simulink model "PerceptionAndGuidance"  (R2026b)
settings: Solver=ode3  StopTime=TFinal
PreLoadFcn:
  | InitVars;
libraries: simulink x3, visiongeotforms x3, raspberrypiAVlib x2, raspberrypiutilitieslib x2, raspberrypiCommlib x2
settings Model: Creator=The MathWorks, Inc.  LastModifiedBy=Deepak Vishwakarma
settings SolverCC: AutoInsertRateTranBlk=on  PositivePriorityOrder=on
settings OptimizationCC: DifferentSizesBufferReuse=on  EfficientTunableParamExpr=on  EnhancedBackFolding=on  MaxStackSize=200000  OptimizationCustomize=off  OptimizeBlockOrder=speed  PassReuseOutputArgsAs=Individual arguments  RemoveInternalMemoryZeroInit=on  RemoveRootLevelIOMemoryZeroInit=on
settings DebuggingCC: ParameterPrecisionLossMsg=none  ParameterTunabilityLossMsg=error
settings HardwareCC: ProdHWDeviceType=ARM Compatible->ARM Cortex-A (32-bit)  ProdLargestAtomicFloat=Double  ProdLargestAtomicInteger=Long  ProdLongLongMode=on
settings ModelReferenceCC: PropagateVarSize=During execution
settings RTWCC: BuildConfiguration=Faster Runs  Description=Embedded Coder  HardwareBoard=Raspberry Pi  SystemTargetFile=ert.tlc  TLCOptions="-aInlineSetEventsForThisBaseRateFcn=TLC_FALSE -aSuppressMultiTaskScheduler=TLC_FALSE  -aRateBasedStepFcn=0"  TemplateMakefile=ert_default_tmf  Toolchain=GNU GCC RPIUtils
settings CodeAppCC: ForceParamTrailComments=on  IgnoreCustomStorageClasses=off  InsertBlockDesc=on  OperatorAnnotations=on  SFDataObjDesc=on  SimulinkDataObjDesc=on
settings ERTTargetCC: CodeReplacementLibrary=ARM Cortex-A CMSIS  ExtModeIntrfLevel=Level2 - Open  ExtModeMexFile=ext_xcp  ExtModeStaticAlloc=on  SupportVariableSizeSignals=on

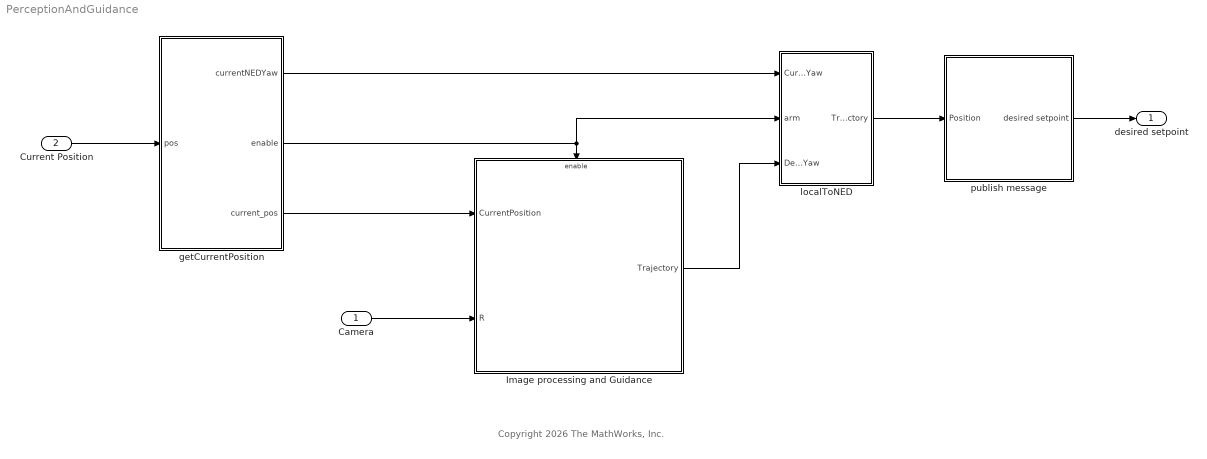
== system PerceptionAndGuidance ==
  note: Copyright 2026 The MathWorks, Inc.
  Camera : Inport
  Current Position : Inport  Port=2
  Image processing and Guidance : Subsystem
  getCurrentPosition : Subsystem  Variant=on
  localToNED : Subsystem
  publish message : Subsystem  Variant=on
  desired setpoint : Outport  OutDataTypeStr=Bus: desiredTargetSetpoints
  wires:
  localToNED/1(Trajectory) -> publish message/1(Position)
  getCurrentPosition/1(currentNEDYaw) -> localToNED/1(CurrentNEDYaw)
  Image processing and Guidance/1(Trajectory) -> localToNED/3(DesiredPosAndYaw)
  getCurrentPosition/2(enable) -> Image processing and Guidance/Enable, localToNED/2(arm)
  Camera/1 -> Image processing and Guidance/2(R)
  Current Position/1 -> getCurrentPosition/1(pos)
  getCurrentPosition/3(current_pos) -> Image processing and Guidance/1(CurrentPosition)
  publish message/1(desired setpoint) -> desired setpoint/1

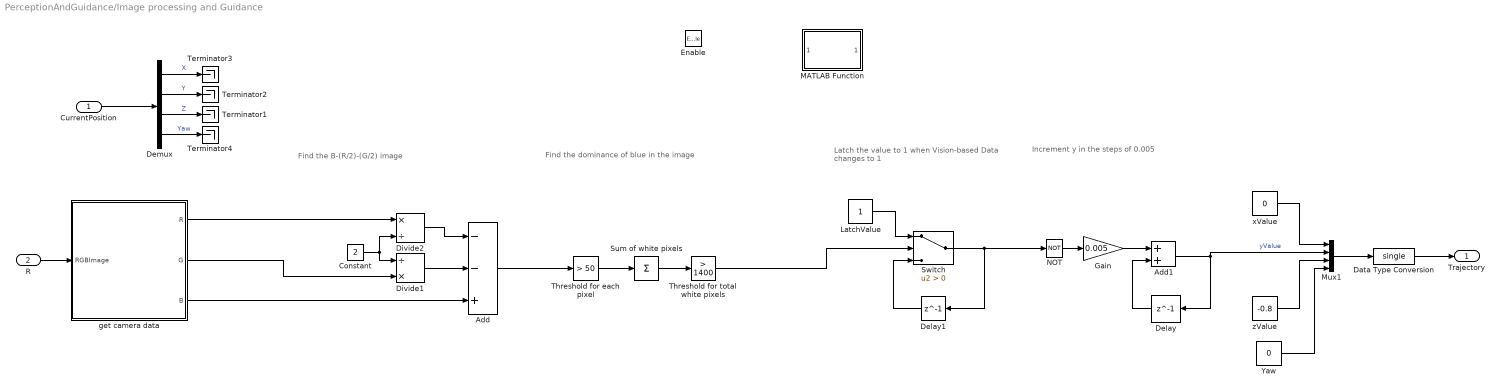
== system PerceptionAndGuidance/Image processing and Guidance ==
  note: Find the dominance of blue in the image
  note: Increment y in the steps of 0.005
  note: Find the B-(R/2)-(G/2) image
  note: Latch the value to 1 when
      | Vision-based Data changes to 1
  CurrentPosition : Inport
  R : Inport  Port=2
  Enable : EnablePort
  Add : Sum  Inputs=--+
  Add1 : Sum
  Constant : Constant  Value=2  SampleTime=-1
  Data Type Conversion : DataTypeConversion  OutDataTypeStr=single  SaturateOnIntegerOverflow=off  RndMeth=Floor
  Delay : Delay  DelayLength=1
  Delay1 : Delay  DelayLength=1
  Demux : Demux
  Divide1 : Product  Inputs=/*
  Divide2 : Product  Inputs=*/
  Gain : Gain  Gain=0.005
  LatchValue : Constant  SampleTime=-1
  MATLAB Function : MATLAB Function  TreatAsAtomicUnit=on
  Mux1 : Mux
  NOT : Logic  Operator=NOT  IconShape=distinctive  AllPortsSameDT=off  OutDataTypeStr=boolean
  Sum of white pixels : Sum  Inputs=+  OutDataTypeStr=uint16
  Switch : Switch  Criteria=u2 > Threshold  SaturateOnIntegerOverflow=off  InputSameDT=off
  Terminator{1..4} (4 alike) : Terminator
  Threshold for each pixel : simulink/Logic and Bit Operations/Compare To Constant  relop=>  const=50  OutDataTypeStr=boolean
  Threshold for total white pixels : simulink/Logic and Bit Operations/Compare To Constant  relop=>  const=1400  OutDataTypeStr=boolean
  Yaw : Constant  Value=0  OutDataTypeStr=double  SampleTime=-1
  get camera data : Subsystem  Variant=on
  xValue : Constant  Value=0  SampleTime=-1
  zValue : Constant  Value=-0.8  SampleTime=-1
  Trajectory : Outport
  wires:
  NOT/1 -> Gain/1
  Divide2/1 -> Add/1
  zValue/1 -> Mux1/3
  Sum of white pixels/1 -> Threshold for total white pixels/1
  get camera data/1(R) -> Divide2/1
  LatchValue/1 -> Switch/1
  Threshold for total white pixels/1 -> Switch/2
  R/1 -> get camera data/1(RGBImage)
  Add1/1 -> Delay/1, Mux1/2  "yValue"
  Constant/1 -> Divide1/1, Divide2/2
  Divide1/1 -> Add/2
  Switch/1 -> NOT/1, Delay1/1
  Delay1/1 -> Switch/3
  Gain/1 -> Add1/1
  Threshold for each pixel/1 -> Sum of white pixels/1
  Delay/1 -> Add1/2
  get camera data/2(G) -> Divide1/2
  Add/1 -> Threshold for each pixel/1
  xValue/1 -> Mux1/1
  get camera data/3(B) -> Add/3
  Data Type Conversion/1 -> Trajectory/1
  Yaw/1 -> Mux1/4
  Mux1/1 -> Data Type Conversion/1
  CurrentPosition/1 -> Demux/1
  Demux/4 -> Terminator4/1  "Yaw"
  Demux/3 -> Terminator1/1  "Z"
  Demux/2 -> Terminator2/1  "Y"
  Demux/1 -> Terminator3/1  "X"

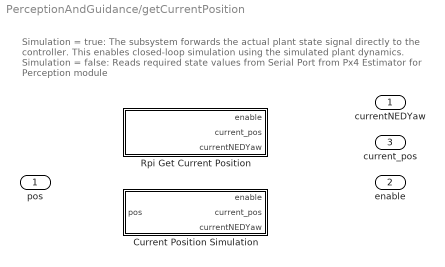
== system PerceptionAndGuidance/getCurrentPosition ==
  note: Simulation = true:
      | The subsystem forwards the actual plant state signal directly to the controller. This enables closed-loop simulation using the simulated plant dynamics.
      |
      | Simulation = false:
      | Reads required state values from Serial Port from Px4 Estimator for Perception module
  pos : Inport  PortDimensions=[1 4]
  Current Position Simulation : Subsystem  VariantControl=Simulation == true
  Rpi Get Current Position : Subsystem  VariantControl=Simulation == false
  currentNEDYaw : Outport
  enable : Outport  Port=2
  current_pos : Outport  Port=3

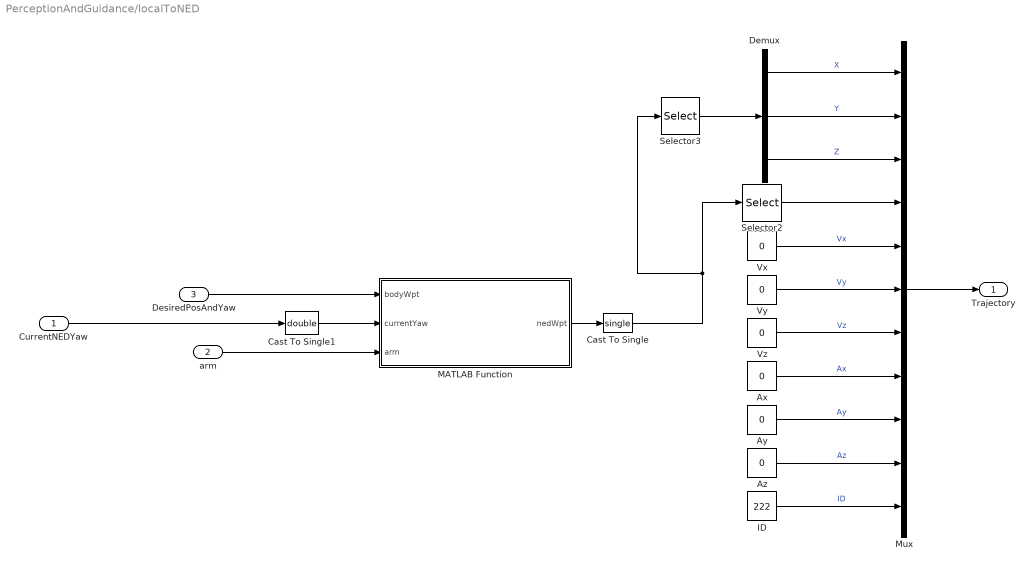
== system PerceptionAndGuidance/localToNED ==
  CurrentNEDYaw : Inport
  arm : Inport  Port=2
  DesiredPosAndYaw : Inport  Port=3
  Ax : Constant  Value=0  OutDataTypeStr=single  SampleTime=-1
  Ay : Constant  Value=0  OutDataTypeStr=single  SampleTime=-1
  Az : Constant  Value=0  OutDataTypeStr=single  SampleTime=-1
  Cast To Single : DataTypeConversion  OutDataTypeStr=single  SaturateOnIntegerOverflow=off  RndMeth=Floor
  Cast To Single1 : DataTypeConversion  OutDataTypeStr=double  SaturateOnIntegerOverflow=off  RndMeth=Floor
  Demux : Demux  Outputs=3
  ID : Constant  Value=222  OutDataTypeStr=single  SampleTime=-1
  MATLAB Function : MATLAB Function  TreatAsAtomicUnit=on
  Mux : Mux  Inputs=11
  Selector2 : Selector  InputPortWidth=4  IndexOptions=Index vector (dialog)  Indices=4  OutputSizes=1
  Selector3 : Selector  InputPortWidth=4  IndexOptions=Index vector (dialog)  Indices=[1:3]  OutputSizes=1
  Vx : Constant  Value=0  OutDataTypeStr=single  SampleTime=-1
  Vy : Constant  Value=0  OutDataTypeStr=single  SampleTime=-1
  Vz : Constant  Value=0  OutDataTypeStr=single  SampleTime=-1
  Trajectory : Outport
  wires:
  Selector3/1 -> Demux/1
  Mux/1 -> Trajectory/1
  Demux/2 -> Mux/2  "Y"
  Demux/3 -> Mux/3  "Z"
  Selector2/1 -> Mux/4
  Cast To Single/1 -> Selector3/1, Selector2/1
  ID/1 -> Mux/11  "ID"
  Demux/1 -> Mux/1  "X"
  Vx/1 -> Mux/5  "Vx"
  Vy/1 -> Mux/6  "Vy"
  Az/1 -> Mux/10  "Az"
  Vz/1 -> Mux/7  "Vz"
  Ay/1 -> Mux/9  "Ay"
  MATLAB Function/1(nedWpt) -> Cast To Single/1
  Ax/1 -> Mux/8  "Ax"
  DesiredPosAndYaw/1 -> MATLAB Function/1(bodyWpt)
  CurrentNEDYaw/1 -> Cast To Single1/1
  Cast To Single1/1 -> MATLAB Function/2(currentYaw)
  arm/1 -> MATLAB Function/3(arm)

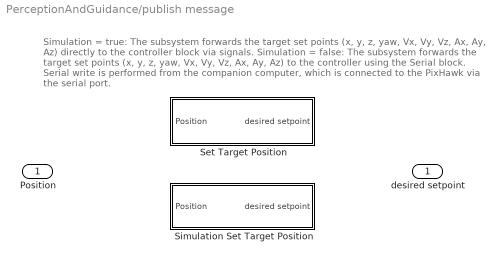
== system PerceptionAndGuidance/publish message ==
  note: Simulation = true:
      | The subsystem forwards the target set points (x, y, z, yaw, Vx, Vy, Vz, Ax, Ay, Az) directly to the controller block via signals.
      |
      | Simulation = false:
      | The subsystem forwards the target set points (x, y, z, yaw, Vx, Vy, Vz, Ax, Ay, Az) to the controller using the Serial block. Serial write is performed from the companion computer, which is connected to the PixHawk via the serial port.
  Position : Inport
  Set Target Position : Subsystem  VariantControl=Simulation == false
  Simulation Set Target Position : Subsystem  VariantControl=Simulation == true
  desired setpoint : Outport

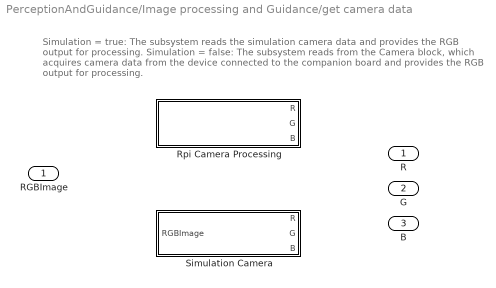
== system PerceptionAndGuidance/Image processing and Guidance/get camera data ==
  note: Simulation = true:
      | The subsystem reads the simulation camera data and provides the RGB output for processing.
      |
      | Simulation = false:
      | The subsystem reads from the Camera block, which acquires camera data from the device connected to the companion board and provides the RGB output for processing.
  RGBImage : Inport  OutDataTypeStr=uint8  PortDimensions=[120, 160, 3]
  Rpi Camera Processing : Subsystem  VariantControl=Simulation == false
  Simulation Camera : Subsystem  VariantControl=Simulation == true
  R : Outport
  G : Outport  Port=2
  B : Outport  Port=3

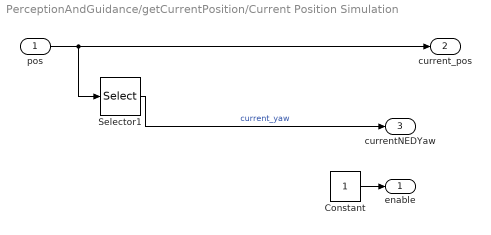
== system PerceptionAndGuidance/getCurrentPosition/Current Position Simulation ==
  pos : Inport
  Constant : Constant  SampleTime=-1
  Selector1 : Selector  InputPortWidth=4  IndexOptions=Index vector (dialog)  Indices=4  OutputSizes=1
  enable : Outport
  current_pos : Outport  Port=2
  currentNEDYaw : Outport  Port=3
  wires:
  pos/1 -> current_pos/1, Selector1/1
  Constant/1 -> enable/1
  Selector1/1 -> currentNEDYaw/1  "current_yaw"

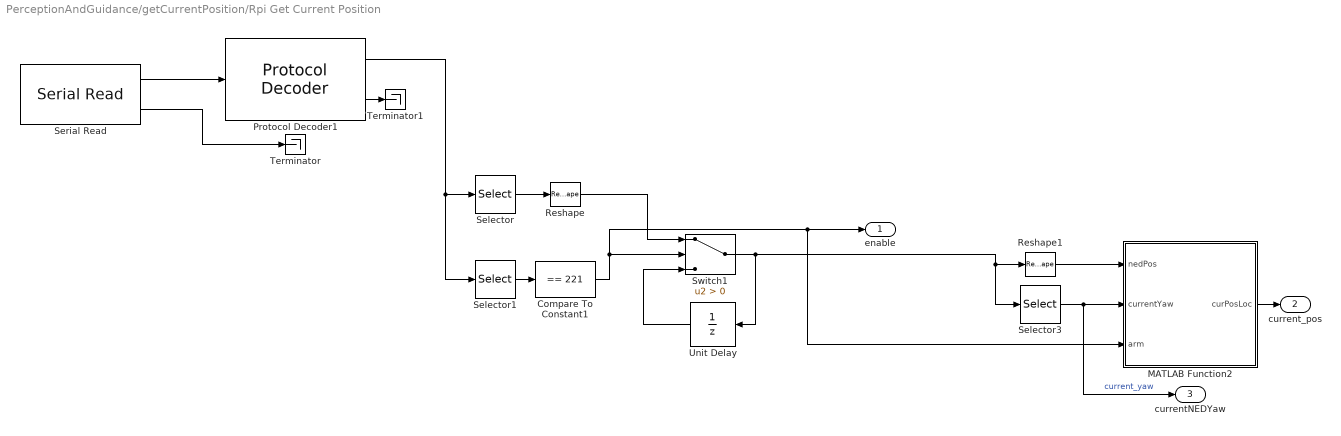
== system PerceptionAndGuidance/getCurrentPosition/Rpi Get Current Position ==
  Compare To Constant1 : simulink/Logic and Bit Operations/Compare To Constant  relop===  const=221  OutDataTypeStr=boolean
  MATLAB Function2 : MATLAB Function  TreatAsAtomicUnit=on
  Protocol Decoder1 : raspberrypiutilitieslib/Protocol Decoder  IsParseCSV=off  Header=[123]  FieldTable={ 'Field1', '5', 'single', 'Little endian' }  IsVariableSizeLastField=off  MaxVariableSizeFieldLength=[]  IsChecksumRequired=off  ChecksumAlgorithm=XOR of bytes  ChecksumSize=[]  TerminatorOption=<none>  CustomTerminatorVal=[]  IsInputLengthAvailable=off
  Reshape : Reshape
  Reshape1 : Reshape  OutputDimensionality=Customize  OutputDimensions=[4,1]
  Selector : Selector  InputPortWidth=5  IndexOptions=Index vector (dialog)  Indices=[1:4]  OutputSizes=1
  Selector1 : Selector  InputPortWidth=5  IndexOptions=Index vector (dialog)  Indices=[5]  OutputSizes=1
  Selector3 : Selector  InputPortWidth=4  IndexOptions=Index vector (dialog)  Indices=4  OutputSizes=1
  Serial Read : raspberrypiCommlib/Serial Read  board=Pi Zero W  SCIModule_=/dev/ttyACM0  Baudrate_=115200  Parity=None  StopBits_=1  HardwareFlowControl=None  ByteOrder=LittleEndian  DataLength=21  DataType=uint8  OutputStatus=on  SampleTime=0.1  blockPlatform=RaspberryPi
  Switch1 : Switch  Criteria=u2 > Threshold  SaturateOnIntegerOverflow=off  InputSameDT=off
  Terminator : Terminator
  Terminator1 : Terminator
  Unit Delay : UnitDelay  InitialCondition=[0 0 0 0]'  SampleTime=-1
  enable : Outport
  current_pos : Outport  Port=2
  currentNEDYaw : Outport  Port=3
  wires:
  Unit Delay/1 -> Switch1/3
  Serial Read/1 -> Protocol Decoder1/1
  Serial Read/2 -> Terminator/1
  Protocol Decoder1/1 -> Selector1/1, Selector/1
  Selector1/1 -> Compare To Constant1/1
  Selector/1 -> Reshape/1
  Reshape/1 -> Switch1/1
  Protocol Decoder1/2 -> Terminator1/1
  Selector3/1 -> currentNEDYaw/1, MATLAB Function2/2(currentYaw)  "current_yaw"
  Compare To Constant1/1 -> MATLAB Function2/3(arm), enable/1, Switch1/2
  Switch1/1 -> Unit Delay/1, Selector3/1, Reshape1/1
  Reshape1/1 -> MATLAB Function2/1(nedPos)
  MATLAB Function2/1(curPosLoc) -> current_pos/1

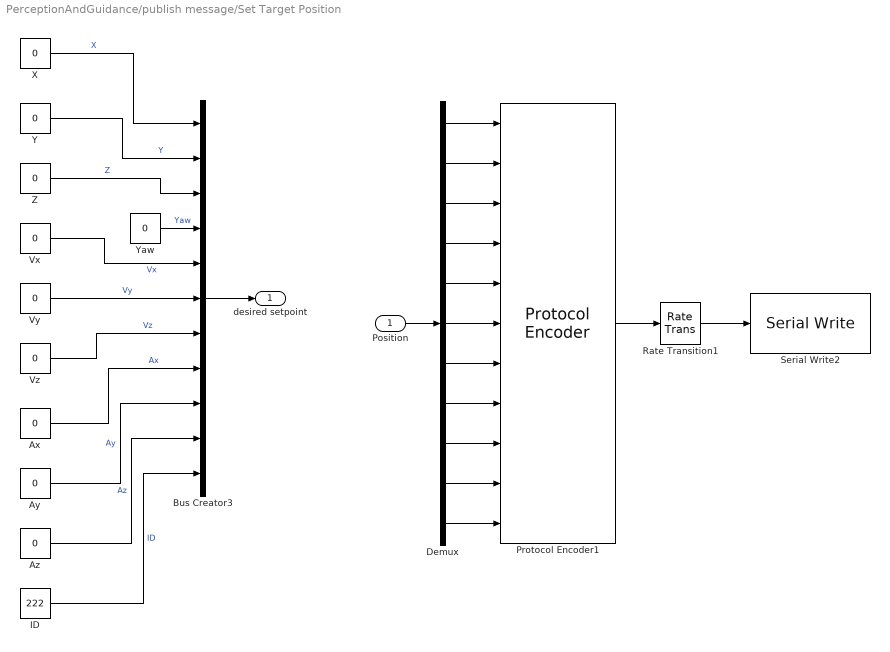
== system PerceptionAndGuidance/publish message/Set Target Position ==
  Position : Inport
  Ax : Constant  Value=0  SampleTime=-1
  Ay : Constant  Value=0  SampleTime=-1
  Az : Constant  Value=0  SampleTime=-1
  Bus Creator3 : BusCreator  Inputs=11  OutDataTypeStr=Bus: desiredTargetSetpoints
  Demux : Demux  Outputs=11
  ID : Constant  Value=222  SampleTime=-1
  Protocol Encoder1 : raspberrypiutilitieslib/Protocol Encoder  Header=[134]  FieldTable={ 'Field1', '1', 'single', 'Little endian'; 'Field2', '1', 'single', 'Little endian'; 'Field3', '1', 'single', 'Little endian'; 'Field4', '1', 'single', 'Little endian'; 'Field5', '1', 'single', 'Little endian'; 'Field6', '1', 'single', 'Little endian'; 'Field7', '1', 'single', 'Little endian'; 'Field8', '1', 'single', 'Little endian'; 'Field9', '1', 'single', 'Little endian'; 'Field10', '1', 'single', 'Little endian'; 'Field11', '1', 'single', 'Little endian' }  IsChecksumRequired=off  ChecksumAlgorithm=XOR of bytes  ChecksumSize=[]  TerminatorOption=<none>  CustomTerminatorVal=[]
  Rate Transition1 : RateTransition  OutPortSampleTime=1/10
  Serial Write2 : raspberrypiCommlib/Serial Write  board=Pi Zero W  SCIModule_=/dev/ttyACM0  Baudrate_=115200  Parity=None  StopBits_=1  HardwareFlowControl=None  ByteOrder=LittleEndian  OutputStatus=off  blockPlatform=RaspberryPi
  Vx : Constant  Value=0  SampleTime=-1
  Vy : Constant  Value=0  SampleTime=-1
  Vz : Constant  Value=0  SampleTime=-1
  X : Constant  Value=0  SampleTime=-1
  Y : Constant  Value=0  SampleTime=-1
  Yaw : Constant  Value=0  SampleTime=-1
  Z : Constant  Value=0  SampleTime=-1
  desired setpoint : Outport  OutDataTypeStr=Bus: desiredTargetSetpoints
  wires:
  Ax/1 -> Bus Creator3/8  "Ax"
  X/1 -> Bus Creator3/1  "X"
  Y/1 -> Bus Creator3/2  "Y"
  Z/1 -> Bus Creator3/3  "Z"
  Ay/1 -> Bus Creator3/9  "Ay"
  Vx/1 -> Bus Creator3/5  "Vx"
  Vy/1 -> Bus Creator3/6  "Vy"
  Vz/1 -> Bus Creator3/7  "Vz"
  Az/1 -> Bus Creator3/10  "Az"
  ID/1 -> Bus Creator3/11  "ID"
  Bus Creator3/1 -> desired setpoint/1
  Rate Transition1/1 -> Serial Write2/1
  Protocol Encoder1/1 -> Rate Transition1/1
  Demux/1 -> Protocol Encoder1/1
  Demux/2 -> Protocol Encoder1/2
  Demux/3 -> Protocol Encoder1/3
  Demux/4 -> Protocol Encoder1/4
  Demux/5 -> Protocol Encoder1/5
  Demux/6 -> Protocol Encoder1/6
  Demux/7 -> Protocol Encoder1/7
  Demux/8 -> Protocol Encoder1/8
  Demux/9 -> Protocol Encoder1/9
  Demux/10 -> Protocol Encoder1/10
  Demux/11 -> Protocol Encoder1/11
  Position/1 -> Demux/1
  Yaw/1 -> Bus Creator3/4  "Yaw"

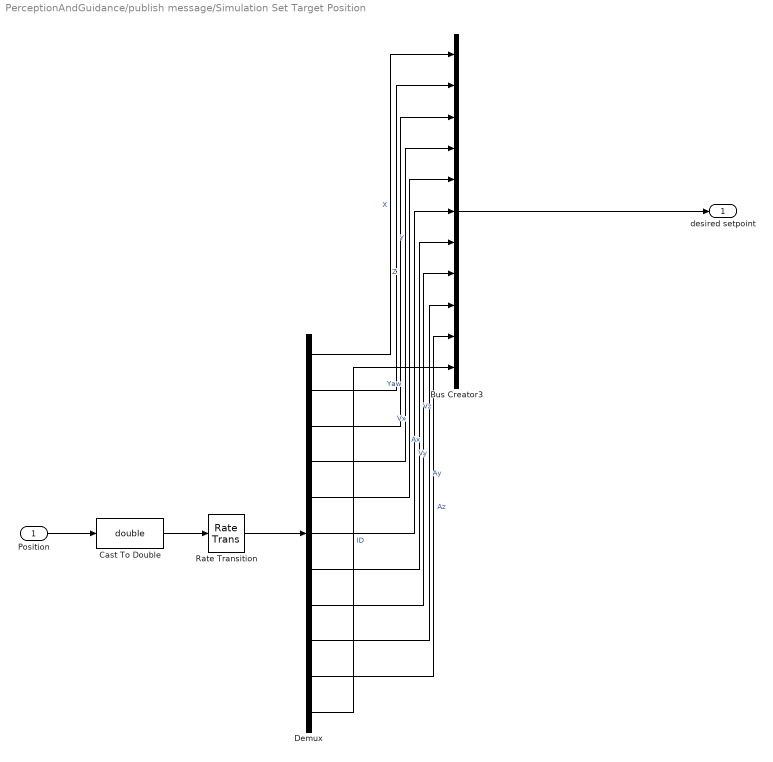
== system PerceptionAndGuidance/publish message/Simulation Set Target Position ==
  Position : Inport
  Bus Creator3 : BusCreator  Inputs=11  OutDataTypeStr=Bus: desiredTargetSetpoints
  Cast To Double : DataTypeConversion  OutDataTypeStr=double  SaturateOnIntegerOverflow=off  RndMeth=Floor
  Demux : Demux  Outputs=11
  Rate Transition : RateTransition  OutPortSampleTime=0.2
  desired setpoint : Outport  OutDataTypeStr=Bus: desiredTargetSetpoints
  wires:
  Demux/1 -> Bus Creator3/1  "X"
  Demux/2 -> Bus Creator3/2  "Y"
  Demux/3 -> Bus Creator3/3  "Z"
  Demux/4 -> Bus Creator3/4  "Yaw"
  Demux/5 -> Bus Creator3/5  "Vx"
  Demux/6 -> Bus Creator3/6  "Vy"
  Demux/7 -> Bus Creator3/7  "Vz"
  Demux/8 -> Bus Creator3/8  "Ax"
  Demux/9 -> Bus Creator3/9  "Ay"
  Demux/10 -> Bus Creator3/10  "Az"
  Demux/11 -> Bus Creator3/11  "ID"
  Position/1 -> Cast To Double/1
  Rate Transition/1 -> Demux/1
  Cast To Double/1 -> Rate Transition/1
  Bus Creator3/1 -> desired setpoint/1

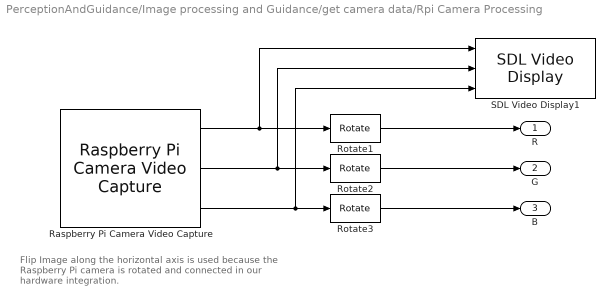
== system PerceptionAndGuidance/Image processing and Guidance/get camera data/Rpi Camera Processing ==
  note: Flip Image along the horizontal axis is used because the Raspberry Pi camera is rotated and connected in our hardware integration.
  Raspberry Pi Camera Video Capture : raspberrypiAVlib/Raspberry Pi Camera Video Capture  CameraNumber=0  Resolution=160x120  CustomResolution=[ 640, 480 ]  PixelFormat=RGB  SampleTime=0.2  HorizontalFlip=on  VerticalFlip=off  ExposureMode=Normal  ExposureCompensation=0.5  MeteringMode=Average  ROI=[ 0.0, 0.0, 1.0, 1.0 ]  Brightness=0.5  Saturation=0.5  Contrast=0.5  Sharpness=0.5  Rotation=0  AWBMode=Auto
  Rotate1 : visiongeotforms/Rotate  outSizeR=Expanded to fit rotated input image  src_angle=Specify via dialog  unit_angle=Degrees  angle=-pi/2  maxAngle=pi  dispImage=Top-left corner  method=Table lookup  fillVal=0  interpMethod=Bilinear  roundingMode=Nearest  overflowMode=on  prodOutputMode=Binary point scaling  prodOutputWordLength=32  prodOutputFracLength=10
  Rotate2 : visiongeotforms/Rotate  outSizeR=Expanded to fit rotated input image  src_angle=Specify via dialog  unit_angle=Degrees  angle=-pi/2  maxAngle=pi  dispImage=Top-left corner  method=Table lookup  fillVal=0  interpMethod=Bilinear  roundingMode=Nearest  overflowMode=on  prodOutputMode=Binary point scaling  prodOutputWordLength=32  prodOutputFracLength=10
  Rotate3 : visiongeotforms/Rotate  outSizeR=Expanded to fit rotated input image  src_angle=Specify via dialog  unit_angle=Degrees  angle=-pi/2  maxAngle=pi  dispImage=Top-left corner  method=Table lookup  fillVal=0  interpMethod=Bilinear  roundingMode=Nearest  overflowMode=on  prodOutputMode=Binary point scaling  prodOutputWordLength=32  prodOutputFracLength=10
  SDL Video Display1 : raspberrypiAVlib/SDL Video Display  title=SDL Video Display  pixelFormat=RGB  pixelOrder=Planar  rowMajor=on  blockPlatform=Raspberry Pi
  R : Outport
  G : Outport  Port=2
  B : Outport  Port=3
  wires:
  Raspberry Pi Camera Video Capture/1 -> SDL Video Display1/1, Rotate1/1
  Raspberry Pi Camera Video Capture/2 -> Rotate2/1, SDL Video Display1/2
  Raspberry Pi Camera Video Capture/3 -> Rotate3/1, SDL Video Display1/3
  Rotate1/1 -> R/1
  Rotate2/1 -> G/1
  Rotate3/1 -> B/1

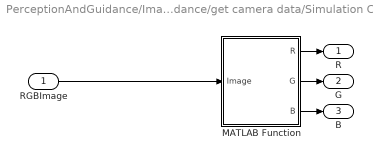
== system PerceptionAndGuidance/Image processing and Guidance/get camera data/Simulation Camera ==
  RGBImage : Inport  OutDataTypeStr=uint8
  MATLAB Function : MATLAB Function  TreatAsAtomicUnit=on
  R : Outport
  G : Outport  Port=2
  B : Outport  Port=3
  wires:
  RGBImage/1 -> MATLAB Function/1(Image)
  MATLAB Function/1(R) -> R/1
  MATLAB Function/2(G) -> G/1
  MATLAB Function/3(B) -> B/1

== matlab function PerceptionAndGuidance/getCurrentPosition/Rpi Get Current Position/MATLAB Function2 ==
  data: nedPos input; curPosLoc output; currentYaw input; arm input
function curPosLoc = ned2body_waypoint(nedPos, currentYaw, arm)
% nedPos: 1x4 [x_ned, y_ned, z, yaw_ned]
% currentYaw: scalar (current yaw from PX4, in radians)
% arm: boolean (true if vehicle is armed)
% Output: 1x4 [x_body, y_body, z, yaw_body]

persistent yaw0 isLatched

if isempty(yaw0)
    yaw0 = single(0);
end
if isempty(isLatched)
    isLatched = false;
end

x_n = nedPos(1);
y_n = nedPos(2);
z_n = nedPos(3);
yaw_n = nedPos(4);

if arm && ~isLatched
    yaw0 = currentYaw;    % latch yaw when arming occurs
    isLatched = true;
elseif ~arm
    isLatched = false;    % reset latch if disarmed
end

if isLatched
    % Transform to body frame relative to yaw0
    x_b =  x_n * cos(yaw0) + y_n * sin(yaw0);
    y_b = -x_n * sin(yaw0) + y_n * cos(yaw0);
    yaw_b = wrapToPi(yaw_n - yaw0);
    curPosLoc = [x_b; y_b; z_n; yaw_b];
else
    % Not armed: just forward readings (no transform)
    curPosLoc = [x_n; y_n; z_n; yaw_n];
end
end

== matlab function PerceptionAndGuidance/Image processing and Guidance/MATLAB Function ==
  data: binaryImg input; centroidX output
function centroidX = findCentroid(binaryImg)
% Calculates horizontal center of mass for detected red pixels
% Input: binaryImg - 2D binary matrix from threshold block

[~, cols] = find(binaryImg);

if ~isempty(cols)
    centroidX = mean(cols); % Average X-coordinate of red pixels
else
    centroidX = size(binaryImg, 2) / 2; % Default to image center if line lost
end
end

== matlab function PerceptionAndGuidance/localToNED/MATLAB Function ==
  data: bodyWpt input; nedWpt output; currentYaw input; arm input
function nedWpt = body2ned_waypoint(bodyWpt, currentYaw, arm)
%#codegen
% Convert body-frame (FRD) waypoint to NED frame
%
% Inputs:
%   bodyWpt:    [x_body, y_body, z, yaw_rel] (4x1 or 1x4)
%               x+ = forward, y+ = right, yaw+ = CW
%               All relative to CURRENT commanded heading
%   currentYaw: scalar, current NED yaw from PX4 feedback (radians)
%   arm:        boolean, true if vehicle is armed
%
% Output:
%   nedWpt: [x_ned, y_ned, z, yaw_ned] in NED frame (4x1)

persistent yaw0 isLatched

if isempty(yaw0)
    yaw0 = double(0);
end
if isempty(isLatched)
    isLatched = false;
end

x_b = bodyWpt(1);
y_b = bodyWpt(2);
z_b = bodyWpt(3);
yaw_rel = bodyWpt(4);

if arm && ~isLatched
    yaw0 = currentYaw;      % latch NED heading at arm time
    isLatched = true;
elseif ~arm
    isLatched = false;
end

if isLatched
    % Full commanded NED heading = initial heading + relative yaw command
    heading_NED = yaw0 + yaw_rel;

    % Rotate body x/y by the full commanded heading
    x_n = x_b * cos(heading_NED) - y_b * sin(heading_NED);
    y_n = x_b * sin(heading_NED) + y_b * cos(heading_NED);

    % Absolute NED yaw (wrapped to [-pi, pi])
    yaw_n = mod(heading_NED + pi, 2*pi) - pi;

    nedWpt = [x_n; y_n; z_b; yaw_n];
else
    nedWpt = [x_b; y_b; z_b; yaw_rel];
end
end

== matlab function PerceptionAndGuidance/Image processing and Guidance/get camera data/Simulation Camera/MATLAB Function ==
  data: Image input; R output; G output; B output
function [R, G, B] = splitRGB(Image)
%#codegen
R = Image(:,:,1);
G = Image(:,:,2);
B = Image(:,:,3);
end
